simulink model "rfdctxrx"  (R2025a)
(part 2 of 7)

      mask TypeOptions t231_DT_dac1_coarse_freq: 0
      mask TypeOptions t231_DT_dac1_nyquist_zone: Zone 1 | Zone 2
      mask TypeOptions t231_DT_dac1_decode_mode: SNR Optimized | Linearity Optimized
      mask TypeOptions t224_adc_clk_src: 224 | 225 | 226 | 227 | 228 | 229 | 230 | 231
      mask TypeOptions t224_clk_dist: None | Input Refclk | PLL Output
      mask TypeOptions t225_adc_clk_src: 224 | 225 | 226 | 227 | 228 | 229 | 230 | 231
      mask TypeOptions t225_clk_dist: None | Input Refclk | PLL Output
      mask TypeOptions t226_adc_clk_src: 224 | 225 | 226 | 227 | 228 | 229 | 230 | 231
      mask TypeOptions t226_clk_dist: None | Input Refclk | PLL Output
      mask TypeOptions t227_adc_clk_src: 224 | 225 | 226 | 227 | 228 | 229 | 230 | 231
      mask TypeOptions t227_clk_dist: None | Input Refclk | PLL Output
      mask TypeOptions t228_dac_clk_src: 224 | 225 | 226 | 227 | 228 | 229 | 230 | 231
      mask TypeOptions t228_clk_dist: None | Input Refclk | PLL Output
      mask TypeOptions t229_dac_clk_src: 224 | 225 | 226 | 227 | 228 | 229 | 230 | 231
      mask TypeOptions t229_clk_dist: None | Input Refclk | PLL Output
      mask TypeOptions t230_dac_clk_src: 224 | 225 | 226 | 227 | 228 | 229 | 230 | 231
      mask TypeOptions t230_clk_dist: None | Input Refclk | PLL Output
      mask TypeOptions t231_dac_clk_src: 224 | 225 | 226 | 227 | 228 | 229 | 230 | 231
      mask TypeOptions t231_clk_dist: None | Input Refclk | PLL Output
      mask DialogControl ADCTileSelect Prompt: ADC Tiles
      mask DialogControl Tile224_container Prompt: Tile 224
      mask DialogControl pll_clocking_config_224 Prompt: Clocking and PLL Configuration
      mask DialogControl t224_QuadTileConfig Prompt: Quad Tile Configuration
      mask DialogControl t224_ADCPair01 Prompt: ADC Pair 0,1
      mask DialogControl t224_QT_adc0 Prompt: ADC 0
      mask DialogControl t224_QT_adc0_DataSettings Prompt: Data Settings
      mask DialogControl t224_QT_adc0_req_axis_clk_label Prompt: Required AXI4-Stream clock:
      mask DialogControl t224_QT_adc0_MixerSettings Prompt: MIxer Settings
      mask DialogControl t224_QT_adc0_AnalogSettings Prompt: Analog Settings
      mask DialogControl t224_QT_adc1 Prompt: ADC 1
      mask DialogControl t224_QT_adc1_DataSettings Prompt: Data Settings
      mask DialogControl t224_QT_adc1_req_axis_clk_label Prompt: Required AXI4-Stream clock:
      mask DialogControl t224_QT_adc1_MixerSettings Prompt: MIxer Settings
      mask DialogControl t224_QT_adc1_AnalogSettings Prompt: Analog Settings
      mask DialogControl ADCPair23 Prompt: ADC Pair 2,3
      mask DialogControl QT_adc2 Prompt: ADC 2
      mask DialogControl t224_QT_adc2_DataSettings Prompt: Data Settings
      mask DialogControl t224_QT_adc2_req_axis_clk_label Prompt: Required AXI4-Stream clock:
      mask DialogControl t224_QT_adc2_MixerSettings Prompt: MIxer Settings
      mask DialogControl t224_QT_adc2_AnalogSettings Prompt: Analog Settings
      mask DialogControl t224_QT_adc3 Prompt: ADC 3
      mask DialogControl t224_QT_adc3_DataSettings Prompt: Data Settings
      mask DialogControl t224_QT_adc3_req_axis_clk_label Prompt: Required AXI4-Stream clock:
      mask DialogControl t224_QT_adc3_MixerSettings Prompt: MIxer Settings
      mask DialogControl t224_QT_adc3_AnalogSettings Prompt: Analog Settings
      mask DialogControl t224_DualTileConfig Prompt: Dual Tile Configuration
      mask DialogControl t224_DT_adc0 Prompt: ADC 0
      mask DialogControl t224_DT_adc0_DataSettings Prompt: Data Settings
      mask DialogControl t224_DT_adc0_req_axis_clk_label Prompt: Required AXI4-Stream clock:
      mask DialogControl t224_DT_adc0_MixerSettings Prompt: MIxer Settings
      mask DialogControl t224_DT_adc0_AnalogSettings Prompt: Analog Settings
      mask DialogControl t224_DT_adc1 Prompt: ADC 1
      mask DialogControl t224_DT_adc1_DataSettings Prompt: Data Settings
      mask DialogControl t224_DT_adc1_req_axis_clk_label Prompt: Required AXI4-Stream clock:
      mask DialogControl t224_DT_adc1_MixerSettings Prompt: MIxer Settings
      mask DialogControl t224_DT_adc1_AnalogSettings Prompt: Analog Settings
      mask DialogControl Tile225_container Prompt: Tile 225
      mask DialogControl pll_clocking_config_225 Prompt: Clocking and PLL Configuration
      mask DialogControl t225_QuadTileConfig Prompt: Quad Tile Configuration
      mask DialogControl t225_ADCPair01 Prompt: ADC Pair 0,1
      mask DialogControl t225_QT_adc0 Prompt: ADC 0
      mask DialogControl t225_QT_adc0_DataSettings Prompt: Data Settings
      mask DialogControl t225_QT_adc0_req_axis_clk_label Prompt: Required AXI4-Stream clock:
      mask DialogControl t225_QT_adc0_MixerSettings Prompt: MIxer Settings
      mask DialogControl t225_QT_adc0_AnalogSettings Prompt: Analog Settings
      mask DialogControl t225_QT_adc1 Prompt: ADC 1
      mask DialogControl t225_QT_adc1_DataSettings Prompt: Data Settings
      mask DialogControl t225_QT_adc1_req_axis_clk_label Prompt: Required AXI4-Stream clock:
      mask DialogControl t225_QT_adc1_MixerSettings Prompt: MIxer Settings
      mask DialogControl t225_QT_adc1_AnalogSettings Prompt: Analog Settings
      mask DialogControl t225_ADCPair23 Prompt: ADC Pair 2,3
      mask DialogControl t225_QT_adc2 Prompt: ADC 2
      mask DialogControl t225_QT_adc2_DataSettings Prompt: Data Settings
      mask DialogControl t225_QT_adc2_req_axis_clk_label Prompt: Required AXI4-Stream clock:
      mask DialogControl t225_QT_adc2_MixerSettings Prompt: MIxer Settings
      mask DialogControl t225_QT_adc2_AnalogSettings Prompt: Analog Settings
      mask DialogControl t225_QT_adc3 Prompt: ADC 3
      mask DialogControl t225_QT_adc3_DataSettings Prompt: Data Settings
      mask DialogControl t225_QT_adc3_req_axis_clk_label Prompt: Required AXI4-Stream clock:
      mask DialogControl t225_QT_adc3_MixerSettings Prompt: MIxer Settings
      mask DialogControl t225_QT_adc3_AnalogSettings Prompt: Analog Settings
      mask DialogControl t225_DualTileConfig Prompt: Dual Tile Configuration
      mask DialogControl t225_DT_adc0 Prompt: ADC 0
      mask DialogControl t225_DT_adc0_DataSettings Prompt: Data Settings
      mask DialogControl t225_DT_adc0_req_axis_clk_label Prompt: Required AXI4-Stream clock:
      mask DialogControl t225_DT_adc0_MixerSettings Prompt: MIxer Settings
      mask DialogControl t225_DT_adc0_AnalogSettings Prompt: Analog Settings
      mask DialogControl t225_DT_adc1 Prompt: ADC 1
      mask DialogControl t225_DT_adc1_DataSettings Prompt: Data Settings
      mask DialogControl t225_DT_adc1_req_axis_clk_label Prompt: Required AXI4-Stream clock:
      mask DialogControl t225_DT_adc1_MixerSettings Prompt: MIxer Settings
      mask DialogControl t225_DT_adc1_AnalogSettings Prompt: Analog Settings
      mask DialogControl Tile226_container Prompt: Tile 226
      mask DialogControl pll_clocking_config_226 Prompt: Clocking and PLL Configuration
      mask DialogControl t226_QuadTileConfig Prompt: Quad Tile Configuration
      mask DialogControl t226_ADCPair01 Prompt: ADC Pair 0,1
      mask DialogControl t226_QT_adc0 Prompt: ADC 0
      mask DialogControl t226_QT_adc0_DataSettings Prompt: Data Settings
      mask DialogControl t226_QT_adc0_req_axis_clk_label Prompt: Required AXI4-Stream clock:
      mask DialogControl t226_QT_adc0_MixerSettings Prompt: MIxer Settings
      mask DialogControl t226_QT_adc0_AnalogSettings Prompt: Analog Settings
      mask DialogControl t226_QT_adc1 Prompt: ADC 1
      mask DialogControl t226_QT_adc1_DataSettings Prompt: Data Settings
      mask DialogControl t226_QT_adc1_req_axis_clk_label Prompt: Required AXI4-Stream clock:
      mask DialogControl t226_QT_adc1_MixerSettings Prompt: MIxer Settings
      mask DialogControl t226_QT_adc1_AnalogSettings Prompt: Analog Settings
      mask DialogControl t226_ADCPair23 Prompt: ADC Pair 2,3
      mask DialogControl t226_QT_adc2 Prompt: ADC 2
      mask DialogControl t226_QT_adc2_DataSettings Prompt: Data Settings
      mask DialogControl t226_QT_adc2_req_axis_clk_label Prompt: Required AXI4-Stream clock:
      mask DialogControl t226_QT_adc2_MixerSettings Prompt: MIxer Settings
      mask DialogControl t226_QT_adc2_AnalogSettings Prompt: Analog Settings
      mask DialogControl t226_QT_adc3 Prompt: ADC 3
      mask DialogControl t226_QT_adc3_DataSettings Prompt: Data Settings
      mask DialogControl t226_QT_adc3_req_axis_clk_label Prompt: Required AXI4-Stream clock:
      mask DialogControl t226_QT_adc3_MixerSettings Prompt: MIxer Settings
      mask DialogControl t226_QT_adc3_AnalogSettings Prompt: Analog Settings
      mask DialogControl t226_DualTileConfig Prompt: Dual Tile Configuration
      mask DialogControl t226_DT_adc0 Prompt: ADC 0
      mask DialogControl t226_DT_adc0_DataSettings Prompt: Data Settings
      mask DialogControl t226_DT_adc0_req_axis_clk_label Prompt: Required AXI4-Stream clock:
      mask DialogControl t226_DT_adc0_MixerSettings Prompt: MIxer Settings
      mask DialogControl t226_DT_adc0_AnalogSettings Prompt: Analog Settings
      mask DialogControl t226_DT_adc1 Prompt: ADC 1
      mask DialogControl t226_DT_adc1_DataSettings Prompt: Data Settings
      mask DialogControl t226_DT_adc1_req_axis_clk_label Prompt: Required AXI4-Stream clock:
      mask DialogControl t226_DT_adc1_MixerSettings Prompt: MIxer Settings
      mask DialogControl t226_DT_adc1_AnalogSettings Prompt: Analog Settings
      mask DialogControl Tile227_container Prompt: Tile 227
      mask DialogControl pll_clocking_config_227 Prompt: Clocking and PLL Configuration
      mask DialogControl t227_QuadTileConfig Prompt: Quad Tile Configuration
      mask DialogControl t227_ADCPair01 Prompt: ADC Pair 0,1
      mask DialogControl t227_QT_adc0 Prompt: ADC 0
      mask DialogControl t227_QT_adc0_DataSettings Prompt: Data Settings
      mask DialogControl t227_QT_adc0_req_axis_clk_label Prompt: Required AXI4-Stream clock:
      mask DialogControl t227_QT_adc0_MixerSettings Prompt: MIxer Settings
      mask DialogControl t227_QT_adc0_AnalogSettings Prompt: Analog Settings
      mask DialogControl t227_QT_adc1 Prompt: ADC 1
      mask DialogControl t227_QT_adc1_DataSettings Prompt: Data Settings
      mask DialogControl t227_QT_adc1_req_axis_clk_label Prompt: Required AXI4-Stream clock:
      mask DialogControl t227_QT_adc1_MixerSettings Prompt: MIxer Settings
      mask DialogControl t227_QT_adc1_AnalogSettings Prompt: Analog Settings
      mask DialogControl t227_ADCPair23 Prompt: ADC Pair 2,3
      mask DialogControl t227_QT_adc2 Prompt: ADC 2
      mask DialogControl t227_QT_adc2_DataSettings Prompt: Data Settings
      mask DialogControl t227_QT_adc2_req_axis_clk_label Prompt: Required AXI4-Stream clock:
      mask DialogControl t227_QT_adc2_MixerSettings Prompt: MIxer Settings
      mask DialogControl t227_QT_adc2_AnalogSettings Prompt: Analog Settings
      mask DialogControl t227_QT_adc3 Prompt: ADC 3
      mask DialogControl t227_QT_adc3_DataSettings Prompt: Data Settings
      mask DialogControl t227_QT_adc3_req_axis_clk_label Prompt: Required AXI4-Stream clock:
      mask DialogControl t227_QT_adc3_MixerSettings Prompt: MIxer Settings
      mask DialogControl t227_QT_adc3_AnalogSettings Prompt: Analog Settings
      mask DialogControl t227_DualTileConfig Prompt: Dual Tile Configuration
      mask DialogControl t227_DT_adc0 Prompt: ADC 0
      mask DialogControl t227_DT_adc0_DataSettings Prompt: Data Settings
      mask DialogControl t227_DT_adc0_req_axis_clk_label Prompt: Required AXI4-Stream clock:
      mask DialogControl t227_DT_adc0_MixerSettings Prompt: MIxer Settings
      mask DialogControl t227_DT_adc0_AnalogSettings Prompt: Analog Settings
      mask DialogControl t227_DT_adc1 Prompt: ADC 1
      mask DialogControl t227_DT_adc1_DataSettings Prompt: Data Settings
      mask DialogControl t227_DT_adc1_req_axis_clk_label Prompt: Required AXI4-Stream clock:
      mask DialogControl t227_DT_adc1_MixerSettings Prompt: MIxer Settings
      mask DialogControl t227_DT_adc1_AnalogSettings Prompt: Analog Settings
      mask DialogControl DACTileSelect Prompt: DAC Tiles
      mask DialogControl Tile228_container Prompt: Tile 228
      mask DialogControl pll_clocking_config_228 Prompt: Clocking and PLL Configuration
      mask DialogControl t228_QuadTileConfig Prompt: Quad Tile Configuration
      mask DialogControl t228_DACPair01 Prompt: DAC Pair 0,1
      mask DialogControl t228_QT_dac0 Prompt: DAC 0
      mask DialogControl t228_QT_dac0_DataSettings Prompt: Data Settings
      mask DialogControl t228_QT_dac0_req_axis_clk_label Prompt: Required AXI4-Stream clock:
      mask DialogControl t228_QT_dac0_MixerSettings Prompt: MIxer Settings
      mask DialogControl t228_QT_dac0_AnalogSettings Prompt: Analog Settings
      mask DialogControl t228_QT_dac1 Prompt: DAC 1
      mask DialogControl t228_QT_dac1_DataSettings Prompt: Data Settings
      mask DialogControl t228_QT_dac1_req_axis_clk_label Prompt: Required AXI4-Stream clock:
      mask DialogControl t228_QT_dac1_MixerSettings Prompt: MIxer Settings
      mask DialogControl t228_QT_dac1_AnalogSettings Prompt: Analog Settings
      mask DialogControl t228_DACPair23 Prompt: DAC Pair 2,3
      mask DialogControl t228_QT_dac2 Prompt: DAC 2
      mask DialogControl t228_QT_dac2_DataSettings Prompt: Data Settings
      mask DialogControl t228_QT_dac2_req_axis_clk_label Prompt: Required AXI4-Stream clock:
      mask DialogControl t228_QT_dac2_MixerSettings Prompt: MIxer Settings
      mask DialogControl t228_QT_dac2_AnalogSettings Prompt: Analog Settings
      mask DialogControl t228_QT_dac3 Prompt: DAC 3
      mask DialogControl t228_QT_dac3_DataSettings Prompt: Data Settings
      mask DialogControl t228_QT_dac3_req_axis_clk_label Prompt: Required AXI4-Stream clock:
      mask DialogControl t228_QT_dac3_MixerSettings Prompt: MIxer Settings
      mask DialogControl t228_QT_dac3_AnalogSettings Prompt: Analog Settings
      mask DialogControl t228_DualTileConfig Prompt: Dual Tile Configuration
      mask DialogControl t228_DT_dac0 Prompt: DAC 0
      mask DialogControl t228_DT_dac0_DataSettings Prompt: Data Settings
      mask DialogControl t228_DT_dac0_req_axis_clk_label Prompt: Required AXI4-Stream clock:
      mask DialogControl t228_DT_dac0_MixerSettings Prompt: MIxer Settings
      mask DialogControl t228_DT_dac0_AnalogSettings Prompt: Analog Settings
      mask DialogControl t228_DT_dac1 Prompt: DAC 1
      mask DialogControl t228_DT_dac1_DataSettings Prompt: Data Settings
      mask DialogControl t228_DT_dac1_req_axis_clk_label Prompt: Required AXI4-Stream clock:
      mask DialogControl t228_DT_dac1_MixerSettings Prompt: MIxer Settings
      mask DialogControl t228_DT_dac1_AnalogSettings Prompt: Analog Settings
      mask DialogControl Tile229_container Prompt: Tile 229
      mask DialogControl pll_clocking_config_229 Prompt: Clocking and PLL Configuration
      mask DialogControl t229_QuadTileConfig Prompt: Quad Tile Configuration
      mask DialogControl t229_DACPair01 Prompt: DAC Pair 0,1
      mask DialogControl t229_QT_dac0 Prompt: DAC 0
      mask DialogControl t229_QT_dac0_DataSettings Prompt: Data Settings
      mask DialogControl t229_QT_dac0_req_axis_clk_label Prompt: Required AXI4-Stream clock:
      mask DialogControl t229_QT_dac0_MixerSettings Prompt: MIxer Settings
      mask DialogControl t229_QT_dac0_AnalogSettings Prompt: Analog Settings
      mask DialogControl t229_QT_dac1 Prompt: DAC 1
      mask DialogControl t229_QT_dac1_DataSettings Prompt: Data Settings
      mask DialogControl t229_QT_dac1_req_axis_clk_label Prompt: Required AXI4-Stream clock:
      mask DialogControl t229_QT_dac1_MixerSettings Prompt: MIxer Settings
      mask DialogControl t229_QT_dac1_AnalogSettings Prompt: Analog Settings
      mask DialogControl t229_DACPair23 Prompt: DAC Pair 2,3
      mask DialogControl t229_QT_dac2 Prompt: DAC 2
      mask DialogControl t229_QT_dac2_DataSettings Prompt: Data Settings
      mask DialogControl t229_QT_dac2_req_axis_clk_label Prompt: Required AXI4-Stream clock:
      mask DialogControl t229_QT_dac2_MixerSettings Prompt: MIxer Settings
      mask DialogControl t229_QT_dac2_AnalogSettings Prompt: Analog Settings
      mask DialogControl t229_QT_dac3 Prompt: DAC 3
      mask DialogControl t229_QT_dac3_DataSettings Prompt: Data Settings
      mask DialogControl t229_QT_dac3_req_axis_clk_label Prompt: Required AXI4-Stream clock:
      mask DialogControl t229_QT_dac3_MixerSettings Prompt: MIxer Settings
      mask DialogControl t229_QT_dac3_AnalogSettings Prompt: Analog Settings
      mask DialogControl t229_DualTileConfig Prompt: Dual Tile Configuration
      mask DialogControl t229_DT_dac0 Prompt: DAC 0
      mask DialogControl t229_DT_dac0_DataSettings Prompt: Data Settings
      mask DialogControl t229_DT_dac0_req_axis_clk_label Prompt: Required AXI4-Stream clock:
      mask DialogControl t229_DT_dac0_MixerSettings Prompt: MIxer Settings
      mask DialogControl t229_DT_dac0_AnalogSettings Prompt: Analog Settings
      mask DialogControl t229_DT_dac1 Prompt: DAC 1
      mask DialogControl t229_DT_dac1_DataSettings Prompt: Data Settings
      mask DialogControl t229_DT_dac1_req_axis_clk_label Prompt: Required AXI4-Stream clock:
      mask DialogControl t229_DT_dac1_MixerSettings Prompt: MIxer Settings
      mask DialogControl t229_DT_dac1_AnalogSettings Prompt: Analog Settings
      mask DialogControl Tile230_container Prompt: Tile 230
      mask DialogControl pll_clocking_config_230 Prompt: Clocking and PLL Configuration
      mask DialogControl t230_QuadTileConfig Prompt: Quad Tile Configuration
      mask DialogControl t230_DACPair01 Prompt: DAC Pair 0,1
      mask DialogControl t230_QT_dac0 Prompt: DAC 0
      mask DialogControl t230_QT_dac0_DataSettings Prompt: Data Settings
      mask DialogControl t230_QT_dac0_req_axis_clk_label Prompt: Required AXI4-Stream clock:
      mask DialogControl t230_QT_dac0_MixerSettings Prompt: MIxer Settings
      mask DialogControl t230_QT_dac0_AnalogSettings Prompt: Analog Settings
      mask DialogControl t230_QT_dac1 Prompt: DAC 1
      mask DialogControl t230_QT_dac1_DataSettings Prompt: Data Settings
      mask DialogControl t230_QT_dac1_req_axis_clk_label Prompt: Required AXI4-Stream clock:
      mask DialogControl t230_QT_dac1_MixerSettings Prompt: MIxer Settings
      mask DialogControl t230_QT_dac1_AnalogSettings Prompt: Analog Settings
      mask DialogControl t230_DACPair23 Prompt: DAC Pair 2,3
      mask DialogControl t230_QT_dac2 Prompt: DAC 2
      mask DialogControl t230_QT_dac2_DataSettings Prompt: Data Settings
      mask DialogControl t230_QT_dac2_req_axis_clk_label Prompt: Required AXI4-Stream clock:
      mask DialogControl t230_QT_dac2_MixerSettings Prompt: MIxer Settings
      mask DialogControl t230_QT_dac2_AnalogSettings Prompt: Analog Settings
      mask DialogControl t230_QT_dac3 Prompt: DAC 3
      mask DialogControl t230_QT_dac3_DataSettings Prompt: Data Settings
      mask DialogControl t230_QT_dac3_req_axis_clk_label Prompt: Required AXI4-Stream clock:
      mask DialogControl t230_QT_dac3_MixerSettings Prompt: MIxer Settings
      mask DialogControl t230_QT_dac3_AnalogSettings Prompt: Analog Settings
      mask DialogControl t230_DualTileConfig Prompt: Dual Tile Configuration
      mask DialogControl t230_DT_dac0 Prompt: DAC 0
      mask DialogControl t230_DT_dac0_DataSettings Prompt: Data Settings
      mask DialogControl t230_DT_dac0_req_axis_clk_label Prompt: Required AXI4-Stream clock:
      mask DialogControl t230_DT_dac0_MixerSettings Prompt: MIxer Settings
      mask DialogControl t230_DT_dac0_AnalogSettings Prompt: Analog Settings
      mask DialogControl t230_DT_dac1 Prompt: DAC 1
      mask DialogControl t230_DT_dac1_DataSettings Prompt: Data Settings
      mask DialogControl t230_DT_dac1_req_axis_clk_label Prompt: Required AXI4-Stream clock:
      mask DialogControl t230_DT_dac1_MixerSettings Prompt: MIxer Settings
      mask DialogControl t230_DT_dac1_AnalogSettings Prompt: Analog Settings
      mask DialogControl Tile231_container Prompt: Tile 231
      mask DialogControl pll_clocking_config_231 Prompt: Clocking and PLL Configuration
      mask DialogControl t231_QuadTileConfig Prompt: Quad Tile Configuration
      mask DialogControl t231_DACPair01 Prompt: DAC Pair 0,1
      mask DialogControl t231_QT_dac0 Prompt: DAC 0
      mask DialogControl t231_QT_dac0_DataSettings Prompt: Data Settings
      mask DialogControl t231_QT_dac0_req_axis_clk_label Prompt: Required AXI4-Stream clock:
      mask DialogControl t231_QT_dac0_MixerSettings Prompt: MIxer Settings
      mask DialogControl t231_QT_dac0_AnalogSettings Prompt: Analog Settings
      mask DialogControl t231_QT_dac1 Prompt: DAC 1
      mask DialogControl t231_QT_dac1_DataSettings Prompt: Data Settings
      mask DialogControl t231_QT_dac1_req_axis_clk_label Prompt: Required AXI4-Stream clock:
      mask DialogControl t231_QT_dac1_MixerSettings Prompt: MIxer Settings
      mask DialogControl t231_QT_dac1_AnalogSettings Prompt: Analog Settings
      mask DialogControl t231_DACPair23 Prompt: DAC Pair 2,3
      mask DialogControl t231_QT_dac2 Prompt: DAC 2
      mask DialogControl t231_QT_dac2_DataSettings Prompt: Data Settings
      mask DialogControl t231_QT_dac2_req_axis_clk_label Prompt: Required AXI4-Stream clock:
      mask DialogControl t231_QT_dac2_MixerSettings Prompt: MIxer Settings
      mask DialogControl t231_QT_dac2_AnalogSettings Prompt: Analog Settings
      mask DialogControl t231_QT_dac3 Prompt: DAC 3
      mask DialogControl t231_QT_dac3_DataSettings Prompt: Data Settings
      mask DialogControl t231_QT_dac3_req_axis_clk_label Prompt: Required AXI4-Stream clock:
      mask DialogControl t231_QT_dac3_MixerSettings Prompt: MIxer Settings
      mask DialogControl t231_QT_dac3_AnalogSettings Prompt: Analog Settings
      mask DialogControl t231_DualTileConfig Prompt: Dual Tile Configuration
      mask DialogControl t231_DT_dac0 Prompt: DAC 0
      mask DialogControl t231_DT_dac0_DataSettings Prompt: Data Settings
      mask DialogControl t231_DT_dac0_req_axis_clk_label Prompt: Required AXI4-Stream clock:
      mask DialogControl t231_DT_dac0_MixerSettings Prompt: MIxer Settings
      mask DialogControl t231_DT_dac0_AnalogSettings Prompt: Analog Settings
      mask DialogControl t231_DT_dac1 Prompt: DAC 1
      mask DialogControl t231_DT_dac1_DataSettings Prompt: Data Settings
      mask DialogControl t231_DT_dac1_req_axis_clk_label Prompt: Required AXI4-Stream clock:
      mask DialogControl t231_DT_dac1_MixerSettings Prompt: MIxer Settings
      mask DialogControl t231_DT_dac1_AnalogSettings Prompt: Analog Settings
      mask DialogControl SystemClocking Prompt: System Clocking And Real-time Ports
      mask DialogControl ADCClocking Prompt: ADC Tile Clocking
      mask DialogControl t224_clock_config Prompt: ADC Tile 224
      mask DialogControl t225_clock_config Prompt: ADC Tile 225
      mask DialogControl t226_clock_config Prompt: ADC Tile 226
      mask DialogControl t227_clock_config Prompt: ADC Tile 227
      mask DialogControl DACClocking Prompt: DAC Tile Clocking
      mask DialogControl t228_clock_config Prompt: DAC Tile 228
      mask DialogControl t229_clock_config Prompt: DAC Tile 229
      mask DialogControl t230_clock_config Prompt: DAC Tile 230
      mask DialogControl t231_clock_config Prompt: DAC Tile 231
  snapshot_ctrl : Subsystem  Tag=xps:sw_reg  AncestorBlock=xps_library/Memory/software_register  mask(swreg){io_dir=From Processor, io_delay=0, init_val=0, sample_period=1, names=[start], bitwidths=1, bin_pts=0, arith_types=2, sim_port=on, show_format=off}
      mask prompts: io_dir "I/O direction"; io_delay "I/O delay"; init_val "Initial Value"; sample_period "Sample period"; names "Bitfield names [msb...lsb]"; bitwidths "Bitfield widths"; bin_pts "Bitfield binary pts"; arith_types "Bitfield types, ufix=0, fix=1, bool=2"; sim_port "Provide sim input/output?"; show_format "Print format string?"
      mask help: A 32-bit software-accessible register. Can be divided into bitfields of varying widths and types using the fields in the block mask.
      mask init:
      | swreg_init(gcb)
      settings: AttributesFormatString=1input
      mask TypeOptions io_dir: To Processor | From Processor
      mask Callback io_dir:
      | mask_enables = get_param(gcb, 'MaskEnables');
      | mask_names = get_param(gcb, 'MaskNames');
      | if strcmp(get_param(gcb, 'io_dir'), 'To Processor'),
      |     mask_enables{ismember(mask_names, 'sample_period')} = 'off';
      | else
      |     mask_enables{ismember(mask_names, 'sample_period')} = 'on';
      | end
      | set_param(gcb, 'MaskEnables', mask_enables);
      mask DialogControl ParameterTabVar0 Prompt: Setup
  tx_bram : Subsystem  Tag=xps:bram  AncestorBlock=xps_library/Memory/shared_bram  mask{arith_type=Unsigned, addr_width=13, data_width=128, reg_prim_output=off, reg_core_output=off, optimization=Minimum_Area, data_bin_pt=0, init_vals=[0:2^13-1], sample_rate=1}
      mask prompts: arith_type "Output Data Type"; addr_width "Address width"; data_width "Data Width"; reg_prim_output "Register Primitive Output"; reg_core_output "Register Core Output"; data_bin_pt "Data Binary Point"; init_vals "Initial values (simulation only)"; sample_rate "Sample rate"
      mask init:
      | shared_bram_mask;
      mask TypeOptions arith_type: Unsigned | Signed  (2's comp)
      mask TypeOptions data_width: 8 | 16 | 32 | 64 | 128
      mask TypeOptions optimization: Minimum_Area | Low_Power
  tx_enable : Subsystem  Tag=xps:sw_reg  AncestorBlock=xps_library/Memory/software_register  mask(swreg){io_dir=From Processor, io_delay=0, init_val=dec2hex(0), sample_period=1, names=reg, bitwidths=1, bin_pts=0, arith_types=2, sim_port=on, show_format=on}
      mask prompts: io_dir "I/O direction"; io_delay "I/O delay"; init_val "Initial Value"; sample_period "Sample period"; names "Bitfield names [msb...lsb]"; bitwidths "Bitfield widths"; bin_pts "Bitfield binary pts"; arith_types "Bitfield types, ufix=0, fix=1, bool=2"; sim_port "Provide sim input/output?"; show_format "Print format string?"
      mask help: A 32-bit software-accessible register. Can be divided into bitfields of varying widths and types using the fields in the block mask.
      mask init:
      | swreg_init(gcb)
      settings: AttributesFormatString=1input:b = 1 bits
      mask TypeOptions io_dir: To Processor | From Processor
      mask Callback io_dir:
      | mask_enables = get_param(gcb, 'MaskEnables');
      | mask_names = get_param(gcb, 'MaskNames');
      | if strcmp(get_param(gcb, 'io_dir'), 'To Processor'),
      |     mask_enables{ismember(mask_names, 'sample_period')} = 'off';
      | else
      |     mask_enables{ismember(mask_names, 'sample_period')} = 'on';
      | end
      | set_param(gcb, 'MaskEnables', mask_enables);
      mask DialogControl ParameterTabVar0 Prompt: Setup
  tx_len : Subsystem  Tag=xps:sw_reg  AncestorBlock=xps_library/Memory/software_register  mask(swreg){io_dir=To Processor, io_delay=0, init_val=dec2hex(0), sample_period=1, names=reg, bitwidths=13, bin_pts=0, arith_types=0, sim_port=on, show_format=on}
      mask prompts: io_dir "I/O direction"; io_delay "I/O delay"; init_val "Initial Value"; sample_period "Sample period"; names "Bitfield names [msb...lsb]"; bitwidths "Bitfield widths"; bin_pts "Bitfield binary pts"; arith_types "Bitfield types, ufix=0, fix=1, bool=2"; sim_port "Provide sim input/output?"; show_format "Print format string?"
      mask help: A 32-bit software-accessible register. Can be divided into bitfields of varying widths and types using the fields in the block mask.
      mask init:
      | swreg_init(gcb)
      settings: AttributesFormatString=1output:uf13.0 = 13 bits
      mask TypeOptions io_dir: To Processor | From Processor
      mask Callback io_dir:
      | mask_enables = get_param(gcb, 'MaskEnables');
      | mask_names = get_param(gcb, 'MaskNames');
      | if strcmp(get_param(gcb, 'io_dir'), 'To Processor'),
      |     mask_enables{ismember(mask_names, 'sample_period')} = 'off';
      | else
      |     mask_enables{ismember(mask_names, 'sample_period')} = 'on';
      | end
      | set_param(gcb, 'MaskEnables', mask_enables);
      mask DialogControl ParameterTabVar0 Prompt: Setup
  wires:
  rfdc/1(m00_axis_tdata) -> bitfield_snapshot/1(in_m00)
  Constant/1 -> bitfield_snapshot/3(we)
  edge_detect/1 -> bitfield_snapshot/4(trig)
  tx_bram/1(data_out) -> munge/1(din)
  munge/1(dout) -> rfdc/6(s10_axis_tdata), rfdc/5(s00_axis_tdata)
  Constant2/1 -> Counter/1
  Counter/1 -> tx_len/1(out_reg), tx_bram/1(addr)
  Constant3/1 -> tx_bram/2(data_in)
  Constant4/1 -> tx_bram/3(we)
  tx_enable/1(in_reg) -> Counter/2
  Constant5/1 -> tx_enable/1(sim_1)
  tx_len/1(sim_out_reg) -> Scope/1
  rfdc/2(m01_axis_tdata) -> bitfield_snapshot/2(in_m01)
  Constant1/1 -> snapshot_ctrl/1(sim_1)
  snapshot_ctrl/1(in_start) -> edge_detect/1
